simulink model "MTE484Lab3"  (R2026b)
settings: Solver=VariableStepAuto  StopTime=200
settings Model: Creator=sebastianassuncao  LastModifiedBy=levirogalla
settings RTWCC: GPUComputeCapability=5.0

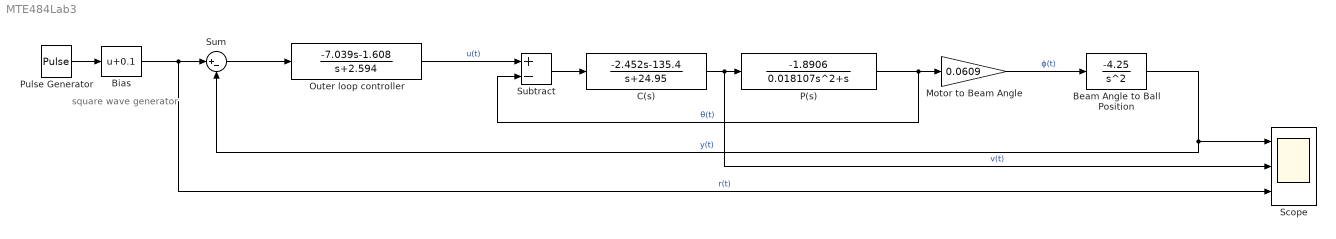
== system MTE484Lab3 ==
  note: square
      | wave
      | generator
  Beam Angle to Ball Position : TransferFcn  Numerator=[-4.25]  Denominator=[1 0 0]
  Bias : Bias  Bias=0.1  SaturateOnIntegerOverflow=off
  C(s) : TransferFcn  Numerator=[-2.452 -135.4]  Denominator=[1 24.95]
  Motor to Beam Angle : Gain  Gain=0.0609
  Outer loop controller : TransferFcn  Numerator=[ -7.039 -1.608]  Denominator=[1 2.594]
  P(s) : TransferFcn  Numerator=[-1.8906]  Denominator=[0.018107 1 0]
  Pulse Generator : DiscretePulseGenerator  PulseType=Time based  Amplitude=0.15  Period=50  PulseWidth=50
  Scope : Scope  NumInputPorts=3
      settings: ActiveDisplayYMinimum=0.14195211418736564  ActiveDisplayYMaximum=0.31832803170946122
  Subtract : Sum  Inputs=+-
  Sum : Sum  Inputs=|+-
  wires:
  P(s)/1 -> Motor to Beam Angle/1, Subtract/2  "θ(t)"
  Subtract/1 -> C(s)/1
  C(s)/1 -> Scope/2, P(s)/1  "v(t)"
  Pulse Generator/1 -> Bias/1
  Outer loop controller/1 -> Subtract/1  "u(t)"
  Bias/1 -> Scope/3, Sum/1  "r(t)"
  Sum/1 -> Outer loop controller/1
  Motor to Beam Angle/1 -> Beam Angle to Ball Position/1  "ϕ(t)"
  Beam Angle to Ball Position/1 -> Scope/1, Sum/2  "y(t)"
